simulink model "Simulacion_NO_Ideal"  (R2026a)
settings: Solver=VariableStepAuto  StopTime=2000
values from neighbouring files (symbols this model uses):
  K = 0.1316    [ControlAnalitico.m]    (also in ModeladoLCA.m = 0.13155478989)
  tau = 166.5    [ControlAnalitico.m]    (also in ModeladoLCA.m = 166.512148502)
libraries: slpidlib x1
settings Model: Creator=magui  LastModifiedBy=Mariano M

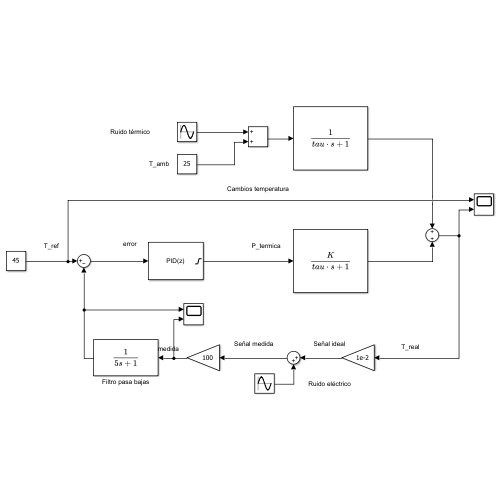
[thumbnail: Simulink's stored preview of the top-level diagram]
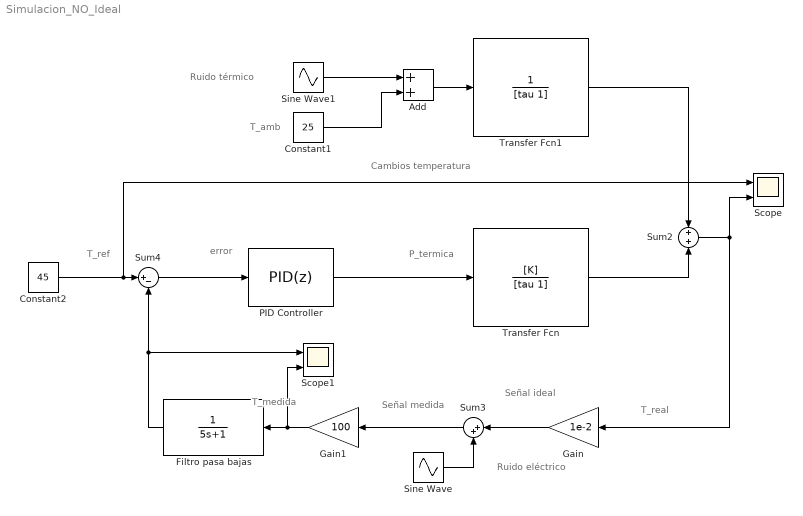
== system Simulacion_NO_Ideal ==
  note: T_amb
  note: P_termica
  note: T_ref
  note: T_real
  note: error
  note: T_medida
  note: Ruido eléctrico
  note: Señal medida
  note: Señal ideal
  note: Cambios temperatura
  note: Ruido térmico
  Add : Sum
  Constant1 : Constant  Value=25
  Constant2 : Constant  Value=45
  Filtro pasa bajas : TransferFcn  Denominator=[5 1]
  Gain : Gain  Gain=1e-2
  Gain1 : Gain  Gain=100
  PID Controller : slpidlib/PID Controller  Controller=PID  Form=Parallel  TimeDomain=Discrete-time  UseExternalTs=off  SampleTime=1  IntegratorMethod=Forward Euler  FilterMethod=Forward Euler  ControllerParametersSource=internal  P=8.43*160  I=0.0506*160  UseKiTs=off  D=0  UseExternalDerivativeSource=off  N=100  UseFilter=on  TunerSelectOption=Transfer Function Based (PID Tuner App)  InitialConditionSource=internal  InitialConditionForIntegrator=0  InitialConditionForFilter=0  DifferentiatorICPrevScaledInput=0  ExternalReset=none  TrackingMode=off  Kt=1  LimitOutput=on  SatLimitsSource=internal  UpperSaturationLimit=160  LowerSaturationLimit=0  LinearizeAsGain=on  AntiWindupMode=back-calculation  Kb=1  LimitIntegrator=off  UpperIntegratorSaturationLimit=inf  LowerIntegratorSaturationLimit=-inf  POutMin=[]  POutMax=[]  IOutMin=[]  IOutMax=[]  DOutMin=[]  DOutMax=[]  NOutMin=[]  NOutMax=[]  SumOutMin=[]  SumOutMax=[]  SaturationOutMin=[]  SaturationOutMax=[]  PParamMin=[]  PParamMax=[]  IParamMin=[]  IParamMax=[]  DParamMin=[]  DParamMax=[]  NParamMin=[]  NParamMax=[]  KbParamMin=[]  KbParamMax=[]  KtParamMin=[]  KtParamMax=[]  KbOutMin=[]  KbOutMax=[]  KtOutMin=[]  KtOutMax=[]  IntegratorOutMin=[]  IntegratorOutMax=[]  FilterOutMin=[]  FilterOutMax=[]  SumI1OutMin=[]  SumI1OutMax=[]  SumI2OutMin=[]  SumI2OutMax=[]  SumI3OutMin=[]  SumI3OutMax=[]  SumI4OutMin=[]  SumI4OutMax=[]  SumDOutMin=[]  SumDOutMax=[]  DifferentiatorOutMin=[]  DifferentiatorOutMax=[]  FilterDiffOutCoefMin=[]  FilterDiffOutCoefMax=[]  ReciprocalOutMin=[]  ReciprocalOutMax=[]  SumDenOutMin=[]  SumDenOutMax=[]  SumNumOutMin=[]  SumNumOutMax=[]  DivideOutMin=[]  DivideOutMax=[]  UdiffTsProdOutMin=[]  UdiffTsProdOutMax=[]  NTsProdOutMin=[]  NTsProdOutMax=[]  UintegralTsProdOutMin=[]  UintegralTsProdOutMax=[]  UngainTsProdOutMin=[]  UngainTsProdOutMax=[]  ClampingZeroOutDataTypeStr=Inherit: Inherit via back propagation  ClampingZeroOutMin=[]  ClampingZeroOutMax=[]  FilterDenConstantOutDataTypeStr=Inherit: Inherit via back propagation  FilterDenConstantOutMin=[]  FilterDenConstantOutMax=[]  PCopyOutDataTypeStr=Inherit: Inherit via back propagation  PCopyOutMin=[]  PCopyOutMax=[]  NCopyOutDataTypeStr=Inherit: Inherit via back propagation  NCopyOutMin=[]  NCopyOutMax=[]  IntegratorContinuousStateAttributes=''  IntegratorStateMustResolveToSignalObject=off  IntegratorRTWStateStorageClass=Auto  FilterContinuousStateAttributes=''  FilterStateMustResolveToSignalObject=off  FilterRTWStateStorageClass=Auto  ParallelPVariant=InternalParameters  IdealPVariant=Disabled  IVariant=InternalParameters  DVariant=InternalParameters  IntegratorVariant=Discrete  SatVariant=Enabled  AWVariant=BackCalculation  PCopyVariant=Disabled  TRVariant=Disabled  FdbkBlocksVariant=Forward  IdealPFdbkVariant=Disabled  SatFdbkVariant=Disabled  DerivativeFilterVariant=ForwardEulerFilter  NVariant=InternalParameters  NCopyVariant=Disabled  FilterICVariant=InternalICsFilter  IntegratorICVariant=InternalICs  ExternalResetVariant=Disabled  TRSumVariant=Passthrough  SumFdbkVariant=Disabled  SumVariant=Sum_PID  TsampFilterVariant=InternalTs  TsampNgainVariant=Passthrough  TsampIntegralVariant=Disabled_SignalSpec  ExternalSaturationOutDataTypeStr=Inherit: Same as second input  DerivativeSourceVariant=ErrorSignal  PreIntVariant=InternalPreInt
  Scope : Scope  NumInputPorts=2
      settings: ActiveDisplayYMinimum=-20  ActiveDisplayYMaximum=60
  Scope1 : Scope  NumInputPorts=2
      settings: ActiveDisplayYMinimum=32.85836  ActiveDisplayYMaximum=44.13196
  Sine Wave : Sin  Amplitude=7.5e-3  Frequency=10  SampleTime=0
  Sine Wave1 : Sin  Amplitude=4  Frequency=10e-5  SampleTime=0
  Sum2 : Sum
  Sum3 : Sum  Inputs=|++
  Sum4 : Sum  Inputs=|+-
  Transfer Fcn : TransferFcn  Numerator=[K]  Denominator=[tau 1]
  Transfer Fcn1 : TransferFcn  Denominator=[tau 1]
  wires:
  Sum4/1 -> PID Controller/1
  Sum2/1 -> Gain/1, Scope/2
  Gain/1 -> Sum3/1
  Sum3/1 -> Gain1/1
  Constant2/1 -> Scope/1, Sum4/1
  Transfer Fcn/1 -> Sum2/2
  PID Controller/1 -> Transfer Fcn/1
  Transfer Fcn1/1 -> Sum2/1
  Sine Wave/1 -> Sum3/2
  Filtro pasa bajas/1 -> Scope1/1, Sum4/2
  Gain1/1 -> Scope1/2, Filtro pasa bajas/1
  Sine Wave1/1 -> Add/1
  Add/1 -> Transfer Fcn1/1
  Constant1/1 -> Add/2
